simulink model "longb747"  (R2024b)
settings: Solver=VariableStepAuto  StartTime=0.0  StopTime=120  RelTol=1e-3
values from neighbouring files (symbols this model uses):
  delta_de_test = deg2rad(delta_de_values(k))    [linearization_validity.m]
  q_init = 0    [b747.m]
  theta_init = p.alpharef    [b747.m]
  V_init = 67.394444    [b747.m]
undefined symbols (not defined in the file or in its folder): p, x_trim
libraries: simulink_extras x6
settings Model: PacingRate=0.100000  Creator=adasu  LastModifiedBy=adasu

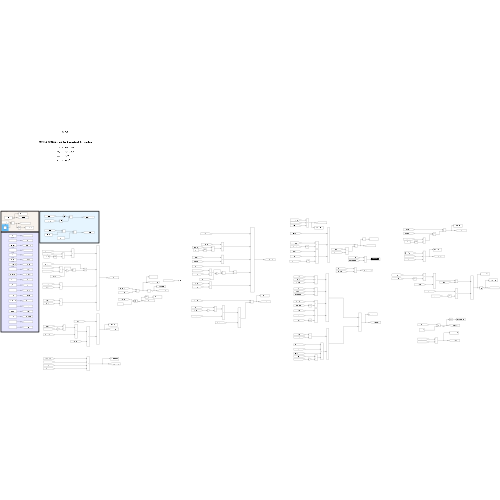
[thumbnail: Simulink's stored preview of the top-level diagram]
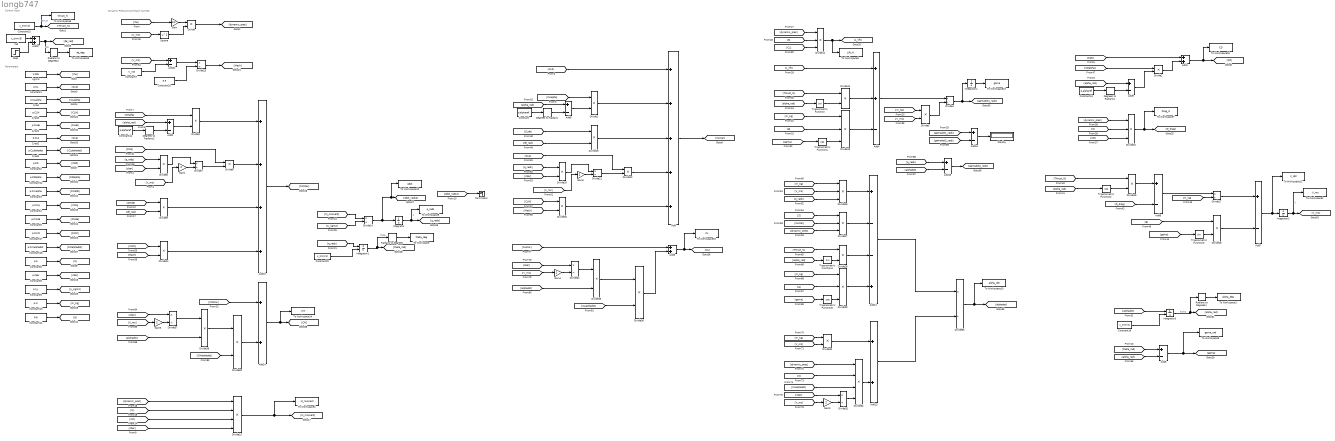
== system longb747 ==
  note: Dynamic Pressure and Mach Number
  note: Control Input
  note: Parameters
  1/rad : Constant  Value=p.CLalpha
  1/rad1 : Constant  Value=p.CLde
  1/rad2 : Constant  Value=p.CLq
  1/rad3 : Constant  Value=p.CLM
  1/rad4 : Constant  Value=p.CLalphadot
  Add : Sum  Inputs=5
  Add{1,3,13..14,17} (5 alike) : Sum
  Add10 : Sum  Inputs=4
  Add{2,5..9,11,15..16} (9 alike) : Sum  Inputs=+-
  Add12 : Sum  Inputs=+--+
  Add4 : Sum  Inputs=++-
  Constant : Constant  Value=p.alpharef
  Constant1 : Constant  Value=p.CL
  Constant10 : Constant  Value=p.m
  Constant11 : Constant  Value=p.g
  Constant12 : Constant  Value=p.CDalpha
  Constant13 : Constant  Value=p.alpharef
  Constant14 : Constant  Value=p.alpharef
  Constant15 : Constant  Value=x_trim(2)
  Constant16 : Constant  Value=p.a
  Constant17 : Constant  Value=p.CmM
  Constant18 : Constant  Value=p.Cmalphadot
  Constant19 : Constant  Value=x_trim(1)
  Constant2 : Constant  Value=p.CD
  Constant20 : Constant  Value=x_trim(1)
  Constant3 : Constant  Value=p.Cmalpha
  Constant4 : Constant  Value=p.Cmq
  Constant5 : Constant  Value=p.Cmde
  Constant6 : Constant  Value=p.S
  Constant7 : Constant  Value=V_init
  Constant8 : Constant  Value=p.cbar
  Constant9 : Constant  Value=p.Iyy
  Degrees to Radians : simulink_extras/Transformations/Degrees to Radians
  Degrees to Radians1 : simulink_extras/Transformations/Degrees to Radians
  Degrees to Radians2 : simulink_extras/Transformations/Degrees to Radians
  Display : Display
  Divide{,1..3,5..6,8..9,12,16,18..20,22,24..25,28,30,35..36,38..39} (22 alike) : Product  Inputs=**
  Divide10 : Product  Inputs=4
  Divide11 : Product  Inputs=3
  Divide{13,15,26..27,29} (5 alike) : Product  Inputs=***
  Divide{4,7,14,17,21,23,31,33..34,37} (10 alike) : Product  Inputs=*/
  Divide32 : Product  Inputs=****
  Gain : Gain  Gain=1/2
  Gain{1..5} (5 alike) : Gain  Gain=2
  Integrator : Integrator  InitialCondition=q_init
  Integrator1 : Integrator  InitialConditionSource=external  InitialCondition=theta_init
  Integrator2 : Integrator  InitialCondition=V_init
  Integrator3 : Integrator  InitialConditionSource=external
  Integrator4 : Integrator
  Radians to Degrees : simulink_extras/Transformations/Radians to Degrees
  Radians to Degrees1 : simulink_extras/Transformations/Radians to Degrees
  Radians to Degrees2 : simulink_extras/Transformations/Radians to Degrees
  Square : Math  Operator=square
  Step : Step  After=delta_de_test  SampleTime=0
  Terminator : Terminator
  To Workspace : ToWorkspace  VariableName=theta_deg  SaveFormat=Timeseries  SampleTime=-1
  To Workspace1 : ToWorkspace  VariableName=alpha_deg  SaveFormat=Timeseries  SampleTime=-1
  To Workspace10 : ToWorkspace  VariableName=alpha_dot  SaveFormat=Timeseries  SampleTime=-1
  To Workspace11 : ToWorkspace  VariableName=V_dot  SaveFormat=Timeseries  SampleTime=-1
  To Workspace12 : ToWorkspace  VariableName=qdot  SaveFormat=Timeseries  SampleTime=-1
  To Workspace13 : ToWorkspace  VariableName=gama  SaveFormat=Timeseries  SampleTime=-1
  To Workspace14 : ToWorkspace  VariableName=Cm  SaveFormat=Timeseries  SampleTime=-1
  To Workspace15 : ToWorkspace  VariableName=CL  SaveFormat=Timeseries  SampleTime=-1
  To Workspace16 : ToWorkspace  VariableName=CD  SaveFormat=Timeseries  SampleTime=-1
  To Workspace2 : ToWorkspace  VariableName=V_ms  SaveFormat=Timeseries  SampleTime=-1
  To Workspace3 : ToWorkspace  VariableName=de_deg  SaveFormat=Timeseries  SampleTime=0.1
  To Workspace4 : ToWorkspace  VariableName=M_moment  SaveFormat=Timeseries  SampleTime=-1
  To Workspace5 : ToWorkspace  VariableName=Lift_N  SaveFormat=Timeseries  SampleTime=-1
  To Workspace6 : ToWorkspace  VariableName=thrust_N  SaveFormat=Timeseries  SampleTime=-1
  To Workspace7 : ToWorkspace  VariableName=Drag_N  SaveFormat=Timeseries  SampleTime=-1
  To Workspace8 : ToWorkspace  VariableName=q_rads  SaveFormat=Timeseries  SampleTime=-1
  To Workspace9 : ToWorkspace  VariableName=gama_rad  SaveFormat=Timeseries  SampleTime=-1
  Trigonometric Function : Trigonometry
  Trigonometric Function1 : Trigonometry  Operator=cos
  Trigonometric Function2 : Trigonometry  Operator=cos
  Trigonometric Function3 : Trigonometry
  Trigonometric Function4 : Trigonometry
  Trigonometric Function5 : Trigonometry  Operator=cos
  kg/m3 : Constant  Value=1.225
  rad : Constant  Value=x_trim(3)
  wires:
  [rho] -> Gain/1
  kg/m3/1 -> [rho]
  [V_ms] -> Square/1
  Gain/1 -> Divide/1
  Square/1 -> Divide/2
  Divide/1 -> [dynamic_pres]
  Constant1/1 -> [CL0]
  1/rad/1 -> [CLalpha]
  Divide1/1 -> Add/2
  [CL0] -> Add/1
  Add/1 -> [CLstar]
  Constant2/1 -> [CD0]
  [CD0] -> Add1/1
  Add1/1 -> To Workspace16/1, [CD]
  Divide6/1 -> Divide7/1
  [V_ms] -> Gain1/1
  Gain1/1 -> Divide7/2
  Divide7/1 -> Divide8/2
  [CMde] -> Divide9/1
  [M_moment] -> Divide14/1
  [Iy_kgm2] -> Divide14/2
  Divide14/1 -> To Workspace12/1, [qdot_rads2], Integrator/1
  Integrator/1 -> To Workspace8/1, [q_rads]  "q"
  [de_rad] -> Divide9/2
  [CMq] -> Divide8/1
  [q_rads] -> Divide6/1
  [cbar] -> Divide6/2
  [q_rads] -> Integrator1/1
  Integrator1/1 -> Radians to Degrees/1, [theta_rad]  "theta"
  [CLalpha] -> Divide1/1
  [S] -> Divide11/2
  [dynamic_pres] -> Divide11/1
  [CL] -> Divide11/3
  Divide11/1 -> To Workspace5/1, [L_lift]
  [alpha_rad] -> Trigonometric Function/1
  Trigonometric Function/1 -> Divide12/2
  [Thrust_N] -> Divide12/1
  Divide12/1 -> Add4/2
  [L_lift] -> Add4/1
  [gama] -> Trigonometric Function1/1
  [m_kg] -> Divide13/1
  [g] -> Divide13/2
  Trigonometric Function1/1 -> Divide13/3
  Divide13/1 -> Add4/3
  [alphadot] -> Integrator3/1
  Integrator3/1 -> Radians to Degrees1/1, [alpha_rad]  "alpha"
  [theta_rad] -> Add5/1
  [alpha_rad] -> Add5/2
  Add5/1 -> To Workspace9/1, [gama]
  [dynamic_pres] -> Divide15/1
  [S] -> Divide15/2
  [CD] -> Divide15/3
  Divide15/1 -> To Workspace7/1, [D_drag]
  [Thrust_N] -> Divide16/1
  [alpha_rad] -> Trigonometric Function2/1
  Trigonometric Function2/1 -> Divide16/2
  Divide16/1 -> Add6/1
  [D_drag] -> Add6/2
  Add6/1 -> Divide17/1
  [m_kg] -> Divide17/2
  [gama] -> Trigonometric Function3/1
  [g] -> Divide18/1
  Trigonometric Function3/1 -> Divide18/2
  Divide17/1 -> Add7/1
  Divide18/1 -> Add7/2
  Add7/1 -> To Workspace11/1, Integrator2/1
  Integrator2/1 -> To Workspace2/1, [V_ms]  "V"
  Constant/1 -> Degrees to Radians/1
  Degrees to Radians/1 -> Add8/2
  [alpha_rad] -> Add8/1
  Add8/1 -> Divide1/2
  Constant3/1 -> [CMalfa]
  Constant4/1 -> [CMq]
  Constant5/1 -> [CMde]
  Constant6/1 -> [S]
  Constant8/1 -> [cbar]
  Constant9/1 -> [Iy_kgm2]
  Constant10/1 -> [m_kg]
  Constant11/1 -> [g]
  Constant12/1 -> [CDalpha]
  [alpha_rad] -> Add9/1
  Degrees to Radians1/1 -> Add9/2
  Constant13/1 -> Degrees to Radians1/1
  [CDalpha] -> Divide2/1
  Add9/1 -> Divide2/2
  Divide2/1 -> Add1/2
  Add2/1 -> Divide3/2
  [alpha_rad] -> Add2/1
  Degrees to Radians2/1 -> Add2/2
  Constant14/1 -> Degrees to Radians2/1
  [CMalfa] -> Divide3/1
  Divide9/1 -> Add10/3
  Divide8/1 -> Add10/2
  Divide3/1 -> Add10/1
  Add10/1 -> [CMstar]
  Constant15/1 -> To Workspace6/1, [Thrust_N]  "thrust"
  [qdot_rads2] -> Terminator/1
  Add4/1 -> Divide4/1
  Divide4/1 -> Integrator4/1, [gamadot1_rads]
  [m_kg] -> Divide5/1
  [V_ms] -> Divide5/2
  Divide5/1 -> Divide4/2
  Radians to Degrees/1 -> To Workspace/1
  1/rad1/1 -> [CLde]
  [CLde] -> Divide19/1
  [de_rad] -> Divide19/2
  Divide19/1 -> Add/3
  1/rad2/1 -> [CLq]
  [cbar] -> Divide20/2
  Divide21/1 -> Divide22/2
  Gain2/1 -> Divide21/2
  [V_ms] -> Gain2/1
  Divide20/1 -> Divide21/1
  [q_rads] -> Divide20/1
  [CLq] -> Divide22/1
  Divide22/1 -> Add/4
  [V_ms] -> Add11/1
  Constant7/1 -> Add11/2
  Add11/1 -> Divide23/1
  Constant16/1 -> Divide23/2
  Divide23/1 -> [Mach]
  1/rad3/1 -> [CLM]
  Constant17/1 -> [CMM]
  [CMM] -> Divide24/1
  Divide24/1 -> Add10/4
  [CLM] -> Divide25/1
  Divide25/1 -> Add/5
  [m_kg] -> Divide26/1
  [V_ms] -> Divide26/2
  [q_rads] -> Divide26/3
  [S] -> Divide27/1
  [CLstar] -> Divide27/2
  [dynamic_pres] -> Divide27/3
  [Thrust_N] -> Divide28/1
  Trigonometric Function4/1 -> Divide28/2
  [alpha_rad] -> Trigonometric Function4/1
  Trigonometric Function5/1 -> Divide29/3
  [g] -> Divide29/2
  [m_kg] -> Divide29/1
  [gama] -> Trigonometric Function5/1
  Divide26/1 -> Add12/1
  Divide27/1 -> Add12/2
  Divide28/1 -> Add12/3
  Divide29/1 -> Add12/4
  [m_kg] -> Divide30/1
  [V_ms] -> Divide30/2
  1/rad4/1 -> [CLalphadot]
  [V_ms] -> Gain3/1
  [cbar] -> Divide31/1
  Gain3/1 -> Divide31/2
  Divide31/1 -> Divide32/4
  [dynamic_pres] -> Divide32/1
  [S] -> Divide32/2
  [CLalphadot] -> Divide32/3
  Divide32/1 -> Add13/2
  Divide30/1 -> Add13/1
  Add12/1 -> Divide33/1
  Add13/1 -> Divide33/2
  Divide33/1 -> To Workspace10/1, [alphadot]
  Radians to Degrees1/1 -> To Workspace1/1
  [V_ms] -> Gain4/1
  Gain4/1 -> Divide34/2
  [cbar] -> Divide34/1
  Divide34/1 -> Divide35/1
  [alphadot] -> Divide35/2
  [CLalphadot] -> Divide36/2
  Divide35/1 -> Divide36/1
  [CLstar] -> Add3/1
  Divide36/1 -> Add3/2
  Add3/1 -> To Workspace15/1, [CL]
  Constant18/1 -> [CMalphadot]
  Divide38/1 -> Divide39/1
  [alphadot] -> Divide38/2
  Divide37/1 -> Divide38/1
  [cbar] -> Divide37/1
  Gain5/1 -> Divide37/2
  [V_ms] -> Gain5/1
  [CMalphadot] -> Divide39/2
  [CMstar] -> Add14/1
  Divide39/1 -> Add14/2
  Add14/1 -> To Workspace14/1, [CM]
  [q_rads] -> Add15/1
  [alphadot] -> Add15/2
  Add15/1 -> [gamadot2_rads]
  [gamadot1_rads] -> Add16/1
  [gamadot2_rads] -> Add16/2
  Add16/1 -> Display/1
  Integrator4/1 -> To Workspace13/1
  Constant19/1 -> Integrator3/2
  Constant20/1 -> Integrator1/2
  Radians to Degrees2/1 -> To Workspace3/1
  [Mach] -> Divide24/2
  [Mach] -> Divide25/2
  [S] -> Divide10/2
  Divide10/1 -> [M_moment], To Workspace4/1
  [cbar] -> Divide10/4
  [dynamic_pres] -> Divide10/1
  [CM] -> Divide10/3
  rad/1 -> Add17/1
  Step/1 -> Add17/2
  Add17/1 -> Radians to Degrees2/1, [de_rad]  "de"
